simulink model "AMC_BLDC"  (R2026a)
settings: configuration reference "AMCBLDC_Configuration" (kept outside this file)
settings Model: DataDictionary=amcbldc.sldd  VariantConfigurationObject=MCVariants  Creator=upattacini  LastModifiedBy=rpumpo
settings ConfigSetRef: SourceName=AMCBLDC_Configuration

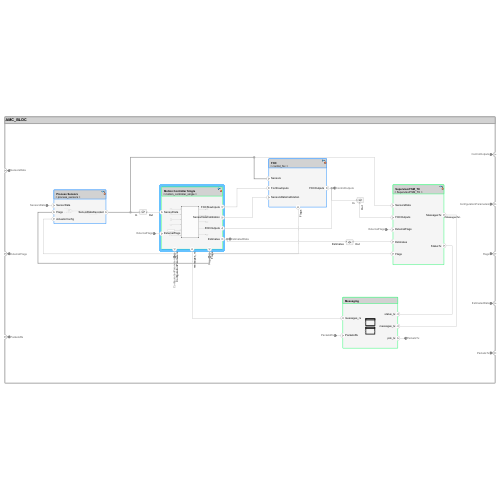
[thumbnail: Simulink's stored preview of the top-level diagram]
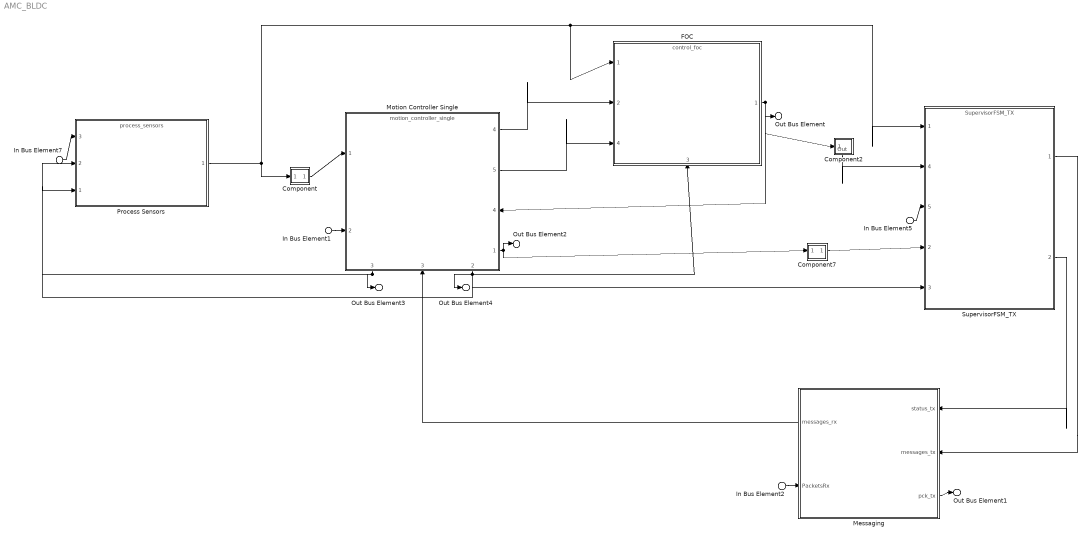
== system AMC_BLDC ==
  In Bus Element7 : Inport  PortName=SensorsData
  In Bus Element1 : Inport  Port=2  PortName=ExternalFlags
  In Bus Element5 : Inport  Port=2  PortName=ExternalFlags
  In Bus Element2 : Inport  Port=3  PortName=PacketsRx
  Component : Subsystem
      settings: PortSchema="{\"entries\":[{\"content\":{\"margin\":10,\"minimumSpacing\":15,\"sides\":[{\"content\":{\"connectorIds\":[\"In1\"]},\"type\":\"ConnectorPlacement.EquallySpacedRectSide\",\"uuid\":\"830d3bb3-c317-4a9d-b479-d4b7625bd8d3\"},{\"content\":{\"connectorIds\":[\"Out1\"],\"side\":\"RIGHT\"},\"type\":\"ConnectorPlacement.EquallySpacedRectSide\",\"uuid\":\"9498d059-e7f6-4620-b5aa-8ea212120189\"},{\"content\":{\"side\":\"TOP\"},\"type\":\"ConnectorPlacement.EquallySpacedRectSide\",\"uuid\":\"e48cad06-2694-4850-bdbf-ad180662e224\"}]},\"type\":\"ConnectorPlacement.EquallySpacedConnector\",\"uuid\":\"6b00e328-32b4-4f3d-a2d8-b512055266a2\"}],\"packageUris\":[\"http://schema.mathworks.com/mf0/Connector/R2020b\"],\"version\":\"1.0\"}"
  Component2 : Subsystem
      settings: PortSchema="{\"entries\":[{\"content\":{\"margin\":10,\"minimumSpacing\":15,\"sides\":[{\"content\":{\"connectorIds\":[\"In1\"]},\"type\":\"ConnectorPlacement.EquallySpacedRectSide\",\"uuid\":\"33e73e3f-3e38-409d-9a68-f5a8c254f44d\"},{\"content\":{\"side\":\"RIGHT\"},\"type\":\"ConnectorPlacement.EquallySpacedRectSide\",\"uuid\":\"3e3f1135-efc4-404f-aae4-c1029426a3e4\"},{\"content\":{\"side\":\"TOP\"},\"type\":\"ConnectorPlacement.EquallySpacedRectSide\",\"uuid\":\"b73facd0-79f3-46e4-b529-4f75d07cbc41\"},{\"content\":{\"connectorIds\":[\"Out1\"],\"side\":\"BOTTOM\"},\"type\":\"ConnectorPlacement.EquallySpacedRectSide\",\"uuid\":\"81ae7ea4-d5aa-4cbc-b0a9-27ede2c6241b\"}]},\"type\":\"ConnectorPlacement.EquallySpacedConnector\",\"uuid\":\"1538baf3-0c35-47d5-a97a-09a81044eaf8\"}],\"packageUris\":[\"http://schema.mathworks.com/mf0/Connector/R2020b\"],\"version\":\"1.0\"}"
  Component7 : Subsystem
      settings: PortSchema="{\"entries\":[{\"content\":{\"margin\":10,\"minimumSpacing\":15,\"sides\":[{\"content\":{\"connectorIds\":[\"In1\"]},\"type\":\"ConnectorPlacement.EquallySpacedRectSide\",\"uuid\":\"830d3bb3-c317-4a9d-b479-d4b7625bd8d3\"},{\"content\":{\"connectorIds\":[\"Out1\"],\"side\":\"RIGHT\"},\"type\":\"ConnectorPlacement.EquallySpacedRectSide\",\"uuid\":\"9498d059-e7f6-4620-b5aa-8ea212120189\"},{\"content\":{\"side\":\"TOP\"},\"type\":\"ConnectorPlacement.EquallySpacedRectSide\",\"uuid\":\"e48cad06-2694-4850-bdbf-ad180662e224\"},{\"content\":{\"side\":\"BOTTOM\"},\"type\":\"ConnectorPlacement.EquallySpacedRectSide\",\"uuid\":\"3c029aad-16f5-4c6f-aa8e-ec60cdf504bb\"}]},\"type\":\"ConnectorPlacement.EquallySpacedConnector\",\"uuid\":\"6b00e328-32b4-4f3d-a2d8-b512055266a2\"}],\"packageUris\":[\"http://schema.mathworks.com/mf0/Connector/R2020b\"],\"version\":\"1.0\"}"
  FOC : ModelReference  ModelNameDialog=control_foc.slx  SimulationMode=Normal  ModelReferenceVersion=10.9
      settings: PortSchema="{\"entries\":[{\"content\":{\"headerSize\":38,\"margin\":15,\"minimumSpacing\":25,\"sides\":[{\"content\":{\"connectorIds\":[\"In1\",\"In2\",\"In4\"]},\"type\":\"ConnectorPlacement.EquallySpacedRectSide\",\"uuid\":\"f5cf413d-ba4f-4573-b6b7-0f383360eb97\"},{\"content\":{\"connectorIds\":[\"Out1\"],\"side\":\"RIGHT\"},\"type\":\"ConnectorPlacement.EquallySpacedRectSide\",\"uuid\":\"fcf07879-e858-44c6-9fd7-a7efb93672a8\"},{\"content\":{\"side\":\"TOP\"},\"type\":\"ConnectorPlacement.EquallySpacedRectSide\",\"uuid\":\"51210f80-623a-465a-bb18-6978a9da34ce\"},{\"content\":{\"connectorIds\":[\"In3\"],\"side\":\"BOTTOM\"},\"type\":\"ConnectorPlacement.EquallySpacedRectSide\",\"uuid\":\"f15bf243-0eb7-466e-91ce-b70aec3f50bc\"}]},\"type\":\"ConnectorPlacement.EquallySpacedConnector\",\"uuid\":\"25ffebdb-746b-4ae0-8cae-cea39d2d3aef\"}],\"packageUris\":[\"http://schema.mathworks.com/mf0/Connector/R2020b\"],\"version\":\"1.0\"}"
  Messaging : Subsystem
      settings: PortSchema="{\"entries\":[{\"content\":{\"headerSize\":26,\"margin\":15,\"minimumSpacing\":25,\"sides\":[{\"content\":{\"connectorIds\":[\"Out2\",\"In1\"]},\"type\":\"ConnectorPlacement.EquallySpacedRectSide\",\"uuid\":\"2148a9ca-a041-4019-8738-bc30807315dc\"},{\"content\":{\"connectorIds\":[\"In3\",\"In2\",\"Out1\"],\"side\":\"RIGHT\"},\"type\":\"ConnectorPlacement.EquallySpacedRectSide\",\"uuid\":\"d2884f22-8c53-43de-b638-02974377300f\"},{\"content\":{\"side\":\"TOP\"},\"type\":\"ConnectorPlacement.EquallySpacedRectSide\",\"uuid\":\"0563c894-934a-48e6-bdf6-cacba4ee5b45\"},{\"content\":{\"side\":\"BOTTOM\"},\"type\":\"ConnectorPlacement.EquallySpacedRectSide\",\"uuid\":\"9d0264c3-5ca4-4a71-92f0-4ebcad17af76\"}]},\"type\":\"ConnectorPlacement.EquallySpacedConnector\",\"uuid\":\"aceedaa9-7f20-49f1-93cc-8d7be38f8964\"}],\"packageUris\":[\"http://schema.mathworks.com/mf0/Connector/R2020b\"],\"version\":\"1.0\"}"
  Motion Controller Single : ModelReference  ModelNameDialog=motion_controller_single.slx  SimulationMode=Normal  ModelReferenceVersion=5.0
      settings: PortSchema="{\"entries\":[{\"content\":{\"headerSize\":38,\"margin\":15,\"minimumSpacing\":25,\"sides\":[{\"content\":{\"connectorIds\":[\"In1\",\"In2\"]},\"type\":\"ConnectorPlacement.EquallySpacedRectSide\",\"uuid\":\"f5cf413d-ba4f-4573-b6b7-0f383360eb97\"},{\"content\":{\"connectorIds\":[\"Out4\",\"Out5\",\"In4\",\"Out1\"],\"side\":\"RIGHT\"},\"type\":\"ConnectorPlacement.EquallySpacedRectSide\",\"uuid\":\"fcf07879-e858-44c6-9fd7-a7efb93672a8\"},{\"content\":{\"side\":\"TOP\"},\"type\":\"ConnectorPlacement.EquallySpacedRectSide\",\"uuid\":\"51210f80-623a-465a-bb18-6978a9da34ce\"},{\"content\":{\"connectorIds\":[\"Out3\",\"In3\",\"Out2\"],\"side\":\"BOTTOM\"},\"type\":\"ConnectorPlacement.EquallySpacedRectSide\",\"uuid\":\"f15bf243-0eb7-466e-91ce-b70aec3f50bc\"}]},\"type\":\"ConnectorPlacement.EquallySpacedConnector\",\"uuid\":\"25ffebdb-746b-4ae0-8cae-cea39d2d3aef\"}],\"packageUris\":[\"http://schema.mathworks.com/mf0/Connector/R2020b\"],\"version\":\"1.0\"}"
  Process Sensors : ModelReference  ModelNameDialog=process_sensors.slx  SimulationMode=Normal  ModelReferenceVersion=2.1
      settings: PortSchema="{\"entries\":[{\"content\":{\"headerSize\":38,\"margin\":15,\"minimumSpacing\":25,\"sides\":[{\"content\":{\"connectorIds\":[\"In3\",\"In2\",\"In1\"]},\"type\":\"ConnectorPlacement.EquallySpacedRectSide\",\"uuid\":\"44154a32-1858-4ed2-962b-d4d560a0fccc\"},{\"content\":{\"connectorIds\":[\"Out1\"],\"side\":\"RIGHT\"},\"type\":\"ConnectorPlacement.EquallySpacedRectSide\",\"uuid\":\"72f5bd24-32be-4e66-8621-cf7439f4e4c3\"},{\"content\":{\"side\":\"TOP\"},\"type\":\"ConnectorPlacement.EquallySpacedRectSide\",\"uuid\":\"6401a363-db3a-40fd-83fa-578661d3700c\"}]},\"type\":\"ConnectorPlacement.EquallySpacedConnector\",\"uuid\":\"41dbb9e1-36eb-448e-a813-87d59e88548a\"}],\"packageUris\":[\"http://schema.mathworks.com/mf0/Connector/R2020b\"],\"version\":\"1.0\"}"
  SupervisorFSM_TX : ModelReference  ModelNameDialog=SupervisorFSM_TX.slx  SimulationMode=Normal  ModelReferenceVersion=11.21
      settings: PortSchema="{\"entries\":[{\"content\":{\"headerSize\":38,\"margin\":15,\"minimumSpacing\":25,\"sides\":[{\"content\":{\"connectorIds\":[\"In1\",\"In4\",\"In5\",\"In2\",\"In3\"]},\"type\":\"ConnectorPlacement.EquallySpacedRectSide\",\"uuid\":\"4aedf767-9c1b-4c88-bc72-7777321bcd41\"},{\"content\":{\"connectorIds\":[\"Out1\",\"Out2\"],\"side\":\"RIGHT\"},\"type\":\"ConnectorPlacement.EquallySpacedRectSide\",\"uuid\":\"aee88cc0-e097-47ae-97af-9ad4a0a9b7bf\"},{\"content\":{\"side\":\"TOP\"},\"type\":\"ConnectorPlacement.EquallySpacedRectSide\",\"uuid\":\"173fabf3-9ac1-4c2f-9d1c-2c077518d79f\"},{\"content\":{\"side\":\"HIDDEN\"},\"type\":\"ConnectorPlacement.EquallySpacedRectSide\",\"uuid\":\"c63b284f-1c4e-4f1a-bde6-4ce5f749d319\"}]},\"type\":\"ConnectorPlacement.EquallySpacedConnector\",\"uuid\":\"40fdf982-cc0d-4196-8efc-330d112bcb29\"}],\"packageUris\":[\"http://schema.mathworks.com/mf0/Connector/R2020b\"],\"version\":\"1.0\"}"
  Out Bus Element : Outport  PortName=ControlOutputs
  Out Bus Element3 : Outport  Port=2  PortName=ConfigurationParameters
  Out Bus Element4 : Outport  Port=3  PortName=Flags
  Out Bus Element2 : Outport  Port=4  PortName=EstimatedData
  Out Bus Element1 : Outport  Port=5  PortName=PacketsTx
  wires:
  In Bus Element2/1 -> Messaging/1(PacketsRx)
  Messaging/1(pck_tx) -> Out Bus Element1/1
  SupervisorFSM_TX/2 -> Messaging/3(status_tx)
  SupervisorFSM_TX/1 -> Messaging/2(messages_tx)
  In Bus Element1/1 -> Motion Controller Single/2
  Messaging/2(messages_rx) -> Motion Controller Single/3
  In Bus Element5/1 -> SupervisorFSM_TX/5
  Motion Controller Single/1 -> Component7/1(Estimates), Out Bus Element2/1
  FOC/1 -> Out Bus Element/1, Motion Controller Single/4, Component2/1(In)
  Motion Controller Single/4 -> FOC/2
  Component2/1(Out) -> SupervisorFSM_TX/4
  Motion Controller Single/3 -> Process Sensors/1, Out Bus Element3/1
  In Bus Element7/1 -> Process Sensors/3
  Motion Controller Single/5 -> FOC/4
  Component7/1(Out) -> SupervisorFSM_TX/2
  Motion Controller Single/2 -> Process Sensors/2, FOC/3, SupervisorFSM_TX/3, Out Bus Element4/1
  Process Sensors/1 -> Component/1(In), SupervisorFSM_TX/1, FOC/1
  Component/1(Out) -> Motion Controller Single/1

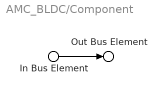
== system AMC_BLDC/Component ==
  In Bus Element : Inport  PortName=In
  Out Bus Element : Outport  PortName=Out
  wires:
  In Bus Element/1 -> Out Bus Element/1

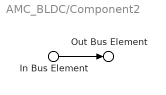
== system AMC_BLDC/Component2 ==
  In Bus Element : Inport  PortName=In
  Out Bus Element : Outport  PortName=Out
  wires:
  In Bus Element/1 -> Out Bus Element/1

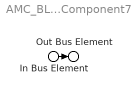
== system AMC_BLDC/Component7 ==
  In Bus Element : Inport  PortName=Estimates
  Out Bus Element : Outport  PortName=Out
  wires:
  In Bus Element/1 -> Out Bus Element/1

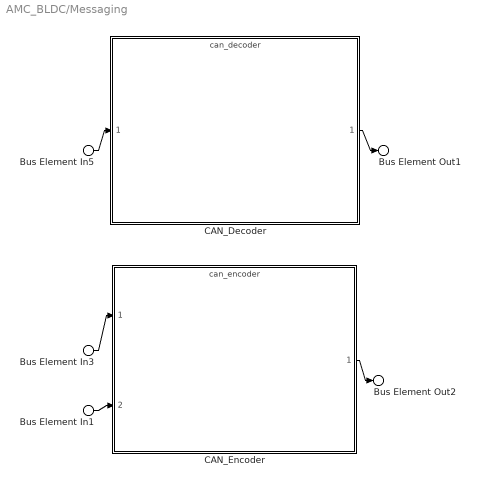
== system AMC_BLDC/Messaging ==
  Bus Element In5 : Inport  PortName=PacketsRx
  Bus Element In3 : Inport  Port=2  PortName=messages_tx
  Bus Element In1 : Inport  Port=3  PortName=status_tx
  CAN_Decoder : ModelReference  ModelNameDialog=can_decoder  SimulationMode=Normal  ModelReferenceVersion=11.0
      settings: PortSchema="{\"entries\":[{\"content\":{\"headerSize\":38,\"margin\":15,\"minimumSpacing\":25,\"sides\":[{\"content\":{\"connectorIds\":[\"In1\"]},\"type\":\"ConnectorPlacement.EquallySpacedRectSide\",\"uuid\":\"b2b94824-c700-4373-91d8-47add34cc094\"},{\"content\":{\"connectorIds\":[\"Out1\"],\"side\":\"RIGHT\"},\"type\":\"ConnectorPlacement.EquallySpacedRectSide\",\"uuid\":\"93c2845f-b99b-4543-8e08-c46ac526332e\"},{\"content\":{\"side\":\"TOP\"},\"type\":\"ConnectorPlacement.EquallySpacedRectSide\",\"uuid\":\"58bbde8c-049b-4e4b-9306-530fa2daad17\"}]},\"type\":\"ConnectorPlacement.EquallySpacedConnector\",\"uuid\":\"2d51588d-c4d7-43f4-87c2-9173ed7811d6\"}],\"packageUris\":[\"http://schema.mathworks.com/mf0/Connector/R2020b\"],\"version\":\"1.0\"}"
  CAN_Encoder : ModelReference  ModelNameDialog=can_encoder  SimulationMode=Normal  ModelReferenceVersion=11.0
      settings: PortSchema="{\"entries\":[{\"content\":{\"headerSize\":38,\"margin\":15,\"minimumSpacing\":25,\"sides\":[{\"content\":{\"connectorIds\":[\"In1\",\"In2\"]},\"type\":\"ConnectorPlacement.EquallySpacedRectSide\",\"uuid\":\"6f4b08cd-f6c5-49bf-b1cb-2cd7d6623be6\"},{\"content\":{\"connectorIds\":[\"Out1\"],\"side\":\"RIGHT\"},\"type\":\"ConnectorPlacement.EquallySpacedRectSide\",\"uuid\":\"50a4d36e-deb5-40a6-b950-d37a57b313ee\"},{\"content\":{\"side\":\"TOP\"},\"type\":\"ConnectorPlacement.EquallySpacedRectSide\",\"uuid\":\"f26608a5-c459-46f7-8e1f-f1e374dcdcf6\"}]},\"type\":\"ConnectorPlacement.EquallySpacedConnector\",\"uuid\":\"e591c604-78a1-48e3-93c5-357c40d96f0b\"}],\"packageUris\":[\"http://schema.mathworks.com/mf0/Connector/R2020b\"],\"version\":\"1.0\"}"
  Bus Element Out2 : Outport  PortName=pck_tx
  Bus Element Out1 : Outport  Port=2  PortName=messages_rx
  wires:
  Bus Element In3/1 -> CAN_Encoder/1
  Bus Element In1/1 -> CAN_Encoder/2
  CAN_Encoder/1 -> Bus Element Out2/1
  Bus Element In5/1 -> CAN_Decoder/1
  CAN_Decoder/1 -> Bus Element Out1/1
